simulink model "FSEA_Vehicle"  (R2026a)
settings: Solver=ode23tb  StopTime=5  FixedStep=.001  RelTol=1e-1
model workspace (MAT data in the model file):
  A_mu = 10
  B_reff = 8.386
  CONVERTER_DATA = [0 0.1 0.2 0.3 0.4 0.5 0.6 0.7 0.8 0.81 0.82 0.83 ... (63 elements, 21x3)]
  Cps = 2
  Cz = 7766.25
  DOWN_TABLE = [0 0 0 0 0 0 5 5 7.5 7.5 15 15 ... (30 elements, 6x5)]
  DOWN_TH_BP = [0 5 40 50 90 100]
  D_reff = 0.25826
  EMAP = [-40 215 245 264 264 267 267 267 267 267 -44 117 ... (110 elements, 10x11)]
  F0z = [6086.4 4324.8]
  F_reff = 0.07394
  F_zmax = 10000
  F_zmin = 100
  F_zo = 4000
  Kz = 48000
  MF : object (value not decoded)
  NCyl = 6
  NE_VEC = [800 1200 1600 2000 2400 2800 3200 3600 4000 4400 4800]
  Pstd = 101325
  Rair = 287
  SUS : object (value not decoded)
  TH_VEC = [0; 20; 30; 40; 50; 60; 70; 80; 90; 100]
  TWAITdn = 1.25
  TWAITup = 0.1
  Tin = [1 2 3 4 5 6 7 8 9 10 2 2 ... (20 elements, 10x2)]
  Tstd = 293.15
  UP_TABLE = [7.5 7.5 15 25 40 40 25 25 35 45 70 80 ... (30 elements, 6x5)]
  UP_TH_BP = [0 25 35 50 90 100]
  VEH : object (value not decoded)
  V_o = 16.7
  V_xlow = 1
  Vd = 0.00346
  WH : object (value not decoded)
  a = 1.515
  alpha_max = 1.5
  alpha_min = -1.5
  b = 1.504
  c_zo = 209651
  epsilon = 0.1
  f_air = [0 0 0 0 0 0 0 0 0 0 0 0 ... (256 elements, 16x16)]
  f_co = [0 0 0 0 0 0 0 0 0 0 0 0 ... (256 elements, 16x16)]
  f_co2 = [0 0 0 0 0 0 0 0 0 0 0 0 ... (256 elements, 16x16)]
  f_eff = [352.135682859 352.135682859 320.724378192 303.655312657 295.930136708 291.240087194 291.240271258 291.240312459 291.240275452 291.240198499 291.240100781 291.240018769 ... (256 elements, 16x16)]
  f_fuel = [0 0 0 0 0 0 0 0 0 0 0 0 ... (256 elements, 16x16)]
  f_hc = [0 0 0 0 0 0 0 0 0 0 0 0 ... (256 elements, 16x16)]
  f_nox = [0 0 0 0 0 0 0 0 0 0 0 0 ... (256 elements, 16x16)]
  f_pm = [0 0 0 0 0 0 0 0 0 0 0 0 ... (256 elements, 16x16)]
  f_susp_axl_bp = [1 2]
  f_susp_dz_bp = [-4 -0.14 -0.13 -0.12 -0.11 -0.1 -0.09 -0.08 -0.07 -0.06 -0.05 -0.04 ... (31 elements, 1x31)]
  f_susp_dzdot_bp = [-4 -0.14 -0.13 -0.12 -0.11 -0.1 -0.09 -0.08 -0.07 -0.06 -0.05 -0.04 ... (31 elements, 1x31)]
  f_susp_fmz = [-213379.591456 -28099.591456 -27619.591456 -27139.591456 -26659.591456 -26179.591456 -25699.591456 -25219.591456 -24739.591456 -24259.591456 -23779.591456 -23299.591456 ... (468968 elements, 31x31x61x2x4)]
  f_susp_geom = [-0.832564012244 0.043269987756 0.045538987756 0.047807987756 0.050076987756 0.052345987756 0.054614987756 0.056883987756 0.059152987756 0.061421987756 0.063690987756 0.065959987756 ... (11346 elements, 31x61x2x3)]
  f_susp_strgdelta_bp = [-0.523598775598 -0.506145483078 -0.488692190558 -0.471238898038 -0.453785605519 -0.436332312999 -0.418879020479 -0.401425727959 -0.383972435439 -0.366519142919 -0.349065850399 -0.331612557879 ... (61 elements, 1x61)]
  f_tbrake = [0 76.8593923996 105.140482948 131.533638111 157.926793274 176.658631717 176.65727296 176.656856686 176.656879077 176.657093756 176.657404516 176.65772406 ... (256 elements, 16x16)]
  f_tbrake_n_bpt = [0 649.519052838 912.419621844 1175.32019085 1438.22075986 1701.12132886 1964.02189787 2226.92246687 2489.82303588 2752.72360489 3015.62417389 3278.5247429 ... (16 elements, 1x16)]
  f_tbrake_t_bpt = [0 34.6410161514 61.0341713143 87.4273264773 113.82048164 140.213636803 166.606791966 192.999947129 219.393102292 245.786257455 272.179412618 298.572567781 ... (16 elements, 1x16)]
  f_texh = [766.752464599 766.752464599 786.17542386 801.679939032 884.591982581 910.574397722 910.571871054 910.570774534 910.570601632 910.570821151 910.571247242 910.571639815 ... (256 elements, 16x16)]
  f_twc_eff_co = [0.17 0.25 0.45 0.99 0.99 0.99 0.99]
  f_twc_eff_hc = [0.21 0.375 0.75 0.98 0.98 0.98 0.98]
  f_twc_eff_lam = [0.909090909 0.944055944 0.979020979 1 1.013986014 1.048951049 1.083916084]
  f_twc_eff_nox = [0.98 0.98 0.98 0.97 0.05 0.02 0]
  h = 0.134
  k_z = 50
  kappa_max = 1.5
  kappa_min = -1.5
  lam_Cx = 1
  lam_Cy = 1
  lam_Cz = 1
  lam_Ex = 1
  lam_Ey = 1
  lam_F_zo = 1
  lam_Hx = 1
  lam_Hy = 1
  lam_Kxkappa = 1
  lam_Kyalpha = 1
  lam_Kygamma = 1
  lam_Kzgamma = 1
  lam_Mr = 1
  lam_Mx = 1
  lam_My = 1
  lam_S = 1
  lam_VMx = 1
  lam_Vx = 1
  lam_Vy = 1
  lam_Vykappa = 1
  lam_muV = 0
  lam_mux = 1
  lam_muy = 1
  lam_t = 1
  lam_xalpha = 1
  lam_ykappa = 1
  numWheel = 4
  p_Cx1 = 1.579
  p_Cy1 = 1.3332
  p_Dx1 = 1.0422
  p_Dx2 = -0.08285
  p_Dx3 = 0
  p_Dy1 = 0.8784
  p_Dy2 = -0.06445
  p_Dy3 = 0
  p_Ex1 = 0.11185
  p_Ex2 = 0.3127
  p_Ex3 = 0
  p_Ex4 = 0.001603
  p_Ey1 = -0.8227
  p_Ey2 = -0.6062
  p_Ey3 = 0.09825
  p_Ey4 = -6.546
  p_Ey5 = 0
  p_Fz1 = 0.7098
  p_Hx1 = 0.00021585
  p_Hx2 = 0.0011538
  p_Hy1 = -0.0018043
  p_Hy2 = 0.003518
  p_Kx1 = 21.69
  p_Kx2 = 13.774
  p_Kx3 = -0.4119
  p_Ky1 = -15.314
  p_Ky2 = 1.7044
  p_Ky3 = 0.36986
  p_Ky4 = 1.9896
  p_Ky5 = 0
  p_Ky6 = -0.9004
  p_Ky7 = -0.2328
  p_Vx1 = 1.5973e-05
  p_Vx2 = 0.0001043
  p_Vy1 = -0.006642
  p_Vy2 = 0.03597
  p_Vy3 = -0.1621
  p_Vy4 = -0.4908
  p_pmx1 = 0
  p_px1 = -0.3489
  p_px2 = 0.382
  p_px3 = -0.09634
  p_px4 = 0.06447
  p_py1 = -0.6249
  p_py2 = -0.06535
  p_py3 = -0.1668
  p_py4 = 0.2834
  p_py5 = 0
  path : object (value not decoded)
  pio = 220000
  q_Fcx = 0
  q_Fz2 = 15.4
  q_Fzy = 0
  q_reo = 0.9974
  q_sx1 = -0.007764
  q_sx10 = 0.2824
  q_sx11 = 5.349
  q_sx12 = 0
  q_sx13 = 0
  q_sx14 = 0
  q_sx2 = 1.1915
  q_sx3 = 0.013948
  q_sx4 = 4.912
  q_sx5 = 1.02
  q_sx6 = 22.83
  q_sx7 = 0.7104
  q_sx8 = -0.023393
  q_sx9 = 0.6581
  q_sy1 = 0.00702
  q_sy2 = 0
  q_sy3 = 0.001515
  q_sy4 = 8.514e-05
  q_sy5 = 0
  q_sy6 = 0
  q_sy7 = 0.9008
  q_sy8 = -0.4089
  q_v1 = 0.0007742
  q_v2 = 0.04667
  r_Bx1 = 12.531
  r_Bx2 = 9.532
  r_Bx3 = 0
  r_By1 = 10.615
  r_By2 = 7.705
  r_By3 = 3.433e-06
  r_By4 = 0
  r_Cx1 = 1.019
  r_Cy1 = 1.0585
  r_Ex1 = -0.4487
  r_Ex2 = -0.4726
  r_Ey1 = 0.3132
  r_Ey2 = 7.63e-06
  r_Hx1 = 0.0002374
  r_Hy1 = 0.011646
  r_Hy2 = 7.63e-06
  r_Vy1 = 0.05654
  r_Vy2 = 7.63e-06
  r_Vy3 = 0
  r_Vy4 = 99.9
  r_Vy5 = 2
  r_Vy6 = 15.814
  r_o = 0.3135
  reqTmaxT = [nan 0.285774810084 0.647179872268 nan nan nan nan nan nan nan nan nan ... (168 elements, 21x8)]
  vehSpd = [0 2.77777777778 5.55555555556 8.33333333333 11.1111111111 13.8888888889 16.6666666667 19.4444444444 22.2222222222 25 27.7777777778 30.5555555556 ... (21 elements, 1x21)]
  vehWidth = 2
  w = 1
symbols that are objects in the model workspace (value not decoded): VEH
undefined symbols (not defined in the file or in its folder): InertFrm
libraries: sharedtransform x6, vehdynlibtirecommon x2, vehdynlibtire x2, autolibutils x2, autolibshared x2
(part 2 of 4)

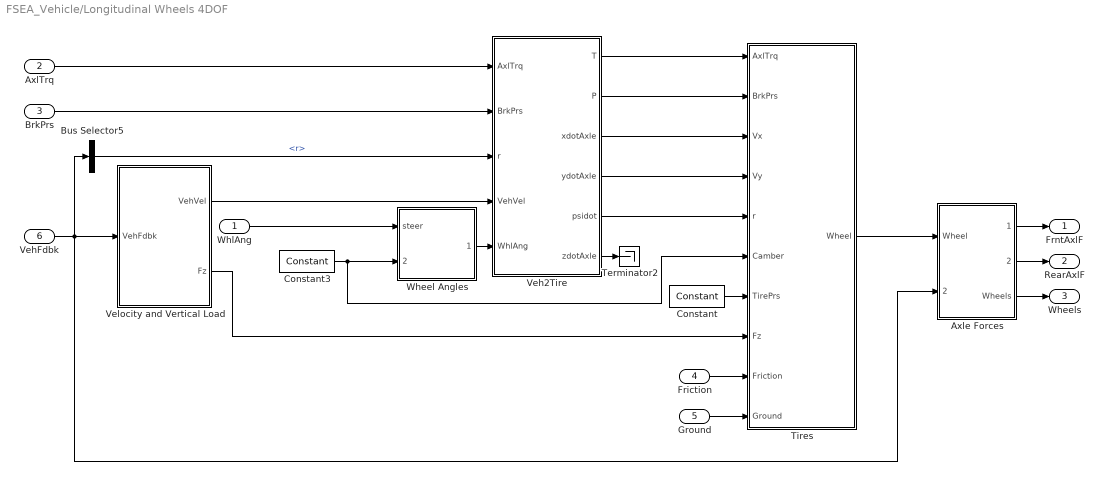
== system FSEA_Vehicle/Longitudinal Wheels 4DOF ==
  WhlAng : Inport
  AxlTrq : Inport  Port=2
  BrkPrs : Inport  Port=3
  Friction : Inport  Port=4  PortDimensions=4
  Ground : Inport  Port=5  PortDimensions=4
  VehFdbk : Inport  Port=6
  Axle Forces : Subsystem  Variant=on  VariantControlMode=label  LabelModeActiveChoice=1
  Bus Selector5 : BusSelector  OutputSignals=BdyFrm.Cg.AngVel.r
  Constant : vehdynlibtirecommon/Constant  const=220000  numWheels=4
  Constant3 : vehdynlibtirecommon/Constant  const=0  numWheels=4
  Terminator2 : Terminator
  Tires : Subsystem  Variant=on  VariantControlMode=label  VariantControl=Choice  LabelModeActiveChoice=0
  Veh2Tire : Subsystem
  Velocity and Vertical Load : Subsystem  Variant=on  VariantControlMode=label  LabelModeActiveChoice=1
  Wheel Angles : Subsystem
  FrntAxlF : Outport  Unit=N  VectorParamsAs1DForOutWhenUnconnected=off
  RearAxlF : Outport  Port=2  Unit=N  VectorParamsAs1DForOutWhenUnconnected=off
  Wheels : Outport  Port=3  VectorParamsAs1DForOutWhenUnconnected=off
  wires:
  Wheel Angles/1(WhlAngB) -> Veh2Tire/5(WhlAng)
  Constant/1 -> Tires/7(TirePrs)
  Constant3/1 -> Wheel Angles/2(camber), Tires/6(Camber)
  Veh2Tire/1(T) -> Tires/1(AxlTrq)
  Veh2Tire/2(P) -> Tires/2(BrkPrs)
  BrkPrs/1 -> Veh2Tire/2(BrkPrs)
  Veh2Tire/6(zdotAxle) -> Terminator2/1
  Veh2Tire/5(psidot) -> Tires/5(r)
  Velocity and Vertical Load/2(Fz) -> Tires/8(Fz)
  Velocity and Vertical Load/1(VehVel) -> Veh2Tire/4(VehVel)
  Axle Forces/1(FrntAxlF) -> FrntAxlF/1
  Axle Forces/2(RearAxlF) -> RearAxlF/1
  Tires/1(Wheel) -> Axle Forces/1(Wheel)
  Axle Forces/3(Wheels) -> Wheels/1
  VehFdbk/1 -> Axle Forces/2(VehFdbk), Bus Selector5/1, Velocity and Vertical Load/1(VehFdbk)
  Ground/1 -> Tires/10(Ground)
  WhlAng/1 -> Wheel Angles/1(steer)
  AxlTrq/1 -> Veh2Tire/1(AxlTrq)
  Friction/1 -> Tires/9(Friction)
  Bus Selector5/1 -> Veh2Tire/3(r)  "<r>"
  Veh2Tire/4(ydotAxle) -> Tires/4(Vy)
  Veh2Tire/3(xdotAxle) -> Tires/3(Vx)

== system FSEA_Vehicle/Vehicle Body 3DOF External Longitudinal Wheels ==
  WhlAng : Inport
  "FwF " : Inport  Port=2
  "FwR " : Inport  Port=3
  WindXYZ : Inport  Port=4
  Bicycle : Subsystem  VariantControl=0
  Dual : Subsystem  VariantControl=1
  " Info" : Outport  VectorParamsAs1DForOutWhenUnconnected=off

== system FSEA_Vehicle/Vehicle Signal Routing ==
  Info : Inport
  Ground : Inport  Port=2
  Dual Track Vehicle Signal Routing : Subsystem  VariantControl=1
  Single Track Vehicle Signal Routing : Subsystem  VariantControl=0
  VehFdbk : Outport

== system FSEA_Vehicle/Longitudinal Wheels 4DOF/Axle Forces ==
  note: 1) Add Subsystem or Model blocks as valid variant choices.
      | 2) You cannot connect blocks at this level. At simulation, connectivity is automatically
      | determined, based on the active variant and port name matching.
  Wheel : Inport
  VehFdbk : Inport  Port=2
  Bicycle : Subsystem  VariantControl=0
  Dual : Subsystem  VariantControl=1
  FrntAxlF : Outport  Unit=N  VectorParamsAs1DForOutWhenUnconnected=off
  RearAxlF : Outport  Port=2  Unit=N  VectorParamsAs1DForOutWhenUnconnected=off
  Wheels : Outport  Port=3

== system FSEA_Vehicle/Longitudinal Wheels 4DOF/Tires ==
  AxlTrq : Inport
  BrkPrs : Inport  Port=2
  Vx : Inport  Port=3
  Vy : Inport  Port=4
  r : Inport  Port=5
  Camber : Inport  Port=6
  TirePrs : Inport  Port=7
  Fz : Inport  Port=8
  Friction : Inport  Port=9
  Ground : Inport  Port=10
  Fiala : Subsystem  VariantControl=1
  MF : Subsystem  VariantControl=0
  Wheel : Outport

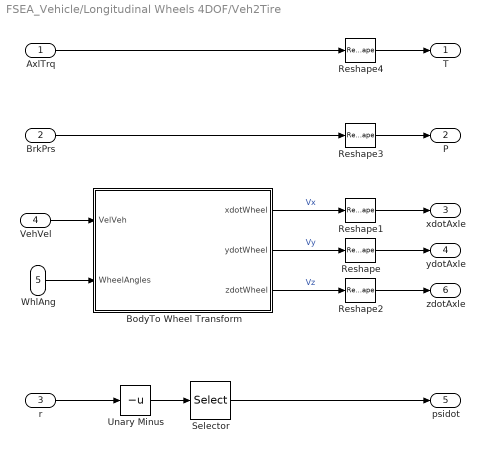
== system FSEA_Vehicle/Longitudinal Wheels 4DOF/Veh2Tire ==
  AxlTrq : Inport
  BrkPrs : Inport  Port=2
  r : Inport  Port=3
  VehVel : Inport  Port=4
  WhlAng : Inport  Port=5
  BodyTo Wheel Transform : Subsystem
  Reshape{,1..4} (5 alike) : Reshape
  Selector : Selector  InputPortWidth=1  IndexOptions=Index vector (dialog)  Indices=[1 1 1 1]  OutputSizes=1
  Unary Minus : UnaryMinus
  T : Outport  VectorParamsAs1DForOutWhenUnconnected=off
  P : Outport  Port=2  VectorParamsAs1DForOutWhenUnconnected=off
  xdotAxle : Outport  Port=3  VectorParamsAs1DForOutWhenUnconnected=off
  ydotAxle : Outport  Port=4  VectorParamsAs1DForOutWhenUnconnected=off
  psidot : Outport  Port=5  VectorParamsAs1DForOutWhenUnconnected=off
  zdotAxle : Outport  Port=6  VectorParamsAs1DForOutWhenUnconnected=off
  wires:
  BrkPrs/1 -> Reshape3/1
  AxlTrq/1 -> Reshape4/1
  BodyTo Wheel Transform/1(xdotWheel) -> Reshape1/1  "Vx"
  BodyTo Wheel Transform/2(ydotWheel) -> Reshape/1  "Vy"
  r/1 -> Unary Minus/1
  Reshape4/1 -> T/1
  VehVel/1 -> BodyTo Wheel Transform/1(VelVeh)
  BodyTo Wheel Transform/3(zdotWheel) -> Reshape2/1  "Vz"
  Unary Minus/1 -> Selector/1
  Reshape3/1 -> P/1
  WhlAng/1 -> BodyTo Wheel Transform/2(WheelAngles)
  Selector/1 -> psidot/1
  Reshape/1 -> ydotAxle/1
  Reshape1/1 -> xdotAxle/1
  Reshape2/1 -> zdotAxle/1

== system FSEA_Vehicle/Longitudinal Wheels 4DOF/Velocity and Vertical Load ==
  note: 1) Add Subsystem or Model blocks as valid variant choices.
      | 2) You cannot connect blocks at this level. At simulation, connectivity is automatically
      | determined, based on the active variant and port name matching.
  VehFdbk : Inport
  Bicycle : Subsystem  VariantControl=0
  Dual : Subsystem  VariantControl=1
  VehVel : Outport  VectorParamsAs1DForOutWhenUnconnected=off
  Fz : Outport  Port=2  PortDimensions=4  VectorParamsAs1DForOutWhenUnconnected=off

== system FSEA_Vehicle/Longitudinal Wheels 4DOF/Wheel Angles ==
  steer : Inport
  camber : Inport  Port=2
  Constant3 : Constant  Value=ones(1,4).*0
  Reshape : Reshape  OutputDimensionality=Row vector (2-D)
  Reshape1 : Reshape  OutputDimensionality=Row vector (2-D)
  Reshape2 : Reshape  OutputDimensionality=Row vector (2-D)
  Vector Concatenate3 : Concatenate  NumInputs=3  Mode=Multidimensional array
  WhlAngB : Outport  VectorParamsAs1DForOutWhenUnconnected=off
  wires:
  camber/1 -> Reshape1/1
  steer/1 -> Reshape/1
  Reshape2/1 -> Vector Concatenate3/2
  Reshape1/1 -> Vector Concatenate3/1
  Constant3/1 -> Reshape2/1
  Reshape/1 -> Vector Concatenate3/3
  Vector Concatenate3/1 -> WhlAngB/1

== system FSEA_Vehicle/Vehicle Body 3DOF External Longitudinal Wheels/Bicycle ==
  "FwF " : Inport
  "FwR " : Inport  Port=2
  WindXYZ : Inport  Port=3
  Terminator{,1..5} (6 alike) : Terminator
  Vehicle Body 3DOF Single Track : autolibshared/Vehicle Body 3DOF Single Track  trackMode=Single (bicycle)  inputMode=External forces  frontSteerMode=off  rearSteerMode=off  extFMode=off  htchFMode=off  extMMode=off  htchMMode=off  windMode=on  extTamb=off  muMode=off  extGndPlnElev=off  extGndPlnRoll=off  extGndPlnPitch=off  extGndPlnDCM=off  extXo=off  extxdoto=off  extYo=off  extydoto=off  extpsio=off  extro=off  aMode=2  NF=VEH.NumberOfWheelsPerAxle  NR=VEH.NumberOfWheelsPerAxle  m=VEH.Mass  a=VEH.FrontAxlePositionfromCG  b=VEH.RearAxlePositionfromCG  h=VEH.HeightCG  dh=1  hh=0.2  X_o=VEH.InitialLongPosition  xdot_o=VEH.InitialLongVel  d=0  hl=0  w=1.922.*[1 1]  CalphaMode=Constant  sigmaMode=on  sigma_f=.1  sigma_r=.1  Cy_f=15000  Cy_r=35000  Cy_f_data=[-9e3 9e3]  alpha_f_brk=[-.1 .1]  Fz_f_brk="[500\t1.555555555555556e+03\t2.611111111111111e+03\t3.666666666666667e+03\t4.722222222222223e+03\t5.777777777777777e+03\t6.833333333333333e+03\t7.888888888888889e+03\t8.944444444444445e+03\t10000]"  Cy_r_data=[-9e3 9e3]  alpha_r_brk=[-.1 .1]  Fz_r_brk="[500\t1.555555555555556e+03\t2.611111111111111e+03\t3.666666666666667e+03\t4.722222222222223e+03\t5.777777777777777e+03\t6.833333333333333e+03\t7.888888888888889e+03\t8.944444444444445e+03\t10000]"  Fznom=3800  Y_o=VEH.InitialLatPosition  ydot_o=VEH.InitialLatVel  Izz=VEH.YawMomentInertia  psi_o=VEH.InitialYawAngle  r_o=VEH.InitialYawRate  Af=VEH.FrontalArea  Cd=.3  Cl=.1  Cpm=.1  beta_w=[0 0.01:0.01:0.3]  Cs=ones(1,31).*0.3  Cym=[0 1e-6:0.01:0.3]  Pabs=101325  Tair=273  g=9.81  mu=1  GndPlnRoll=0  GndPlnPitch=0  GndPlnElev=0  xdot_tol=.1  Fxtire_sat=7e3*1e3  Fytire_sat=2e3*1e3  longOff=0  latOff=0  vertOff=VEH.HeightCG  wrapAng=off
  " Info" : Outport  VectorParamsAs1DForOutWhenUnconnected=off
  wires:
  "FwR "/1 -> Vehicle Body 3DOF Single Track/2
  "FwF "/1 -> Vehicle Body 3DOF Single Track/1
  Vehicle Body 3DOF Single Track/1 -> " Info"/1
  Vehicle Body 3DOF Single Track/6 -> Terminator/1
  Vehicle Body 3DOF Single Track/7 -> Terminator1/1
  WindXYZ/1 -> Vehicle Body 3DOF Single Track/3
  Vehicle Body 3DOF Single Track/4 -> Terminator2/1
  Vehicle Body 3DOF Single Track/5 -> Terminator3/1
  Vehicle Body 3DOF Single Track/2 -> Terminator4/1
  Vehicle Body 3DOF Single Track/3 -> Terminator5/1

== system FSEA_Vehicle/Vehicle Body 3DOF External Longitudinal Wheels/Dual ==
  WhlAng : Inport
  "FwF " : Inport  Port=2
  "FwR " : Inport  Port=3
  WindXYZ : Inport  Port=4
  Selector : Selector  InputPortWidth=4  IndexOptions=Index vector (dialog)  Indices=[1 2]  OutputSizes=1
  Terminator{,1..5} (6 alike) : Terminator
  Vehicle Body 3DOF Dual Track : autolibshared/Vehicle Body 3DOF Single Track  trackMode=Dual  inputMode=External forces  frontSteerMode=on  rearSteerMode=off  extFMode=off  htchFMode=off  extMMode=off  htchMMode=off  windMode=on  extTamb=off  muMode=off  extGndPlnElev=off  extGndPlnRoll=off  extGndPlnPitch=off  extGndPlnDCM=off  extXo=off  extxdoto=off  extYo=off  extydoto=off  extpsio=off  extro=off  aMode=2  NF=VEH.NumberOfWheelsPerAxle  NR=VEH.NumberOfWheelsPerAxle  m=310  a=0.775  b=0.775  h=0.289  dh=1  hh=0.2  X_o=VEH.InitialLongPosition  xdot_o=VEH.InitialLatVel  d=0  hl=0  w=[1.200, 1.150]  CalphaMode=Constant  sigmaMode=on  sigma_f=.1  sigma_r=.1  Cy_f=15000  Cy_r=35000  Cy_f_data=[-9e3 9e3]  alpha_f_brk=[-.1 .1]  Fz_f_brk="[500\t1.555555555555556e+03\t2.611111111111111e+03\t3.666666666666667e+03\t4.722222222222223e+03\t5.777777777777777e+03\t6.833333333333333e+03\t7.888888888888889e+03\t8.944444444444445e+03\t10000]"  Cy_r_data=[-9e3 9e3]  alpha_r_brk=[-.1 .1]  Fz_r_brk="[500\t1.555555555555556e+03\t2.611111111111111e+03\t3.666666666666667e+03\t4.722222222222223e+03\t5.777777777777777e+03\t6.833333333333333e+03\t7.888888888888889e+03\t8.944444444444445e+03\t10000]"  Fznom=3800  Y_o=VEH.InitialLatPosition  ydot_o=VEH.InitialLatVel  Izz=VEH.YawMomentInertia  psi_o=VEH.InitialYawAngle  r_o=VEH.InitialYawRate  Af=1  Cd=.3  Cl=.1  Cpm=.1  beta_w=[0 0.01:0.01:0.3]  Cs=ones(1,31).*0.3  Cym=[0 1e-6:0.001:0.03]  Pabs=101325  Tair=273  g=9.81  mu=1  GndPlnRoll=0  GndPlnPitch=0  GndPlnElev=0  xdot_tol=.01  Fxtire_sat=7e3*1e3  Fytire_sat=2e3*1e3  longOff=0  latOff=0  vertOff=VEH.HeightCG  wrapAng=on
  " Info" : Outport  VectorParamsAs1DForOutWhenUnconnected=off
  wires:
  Vehicle Body 3DOF Dual Track/1 -> " Info"/1
  Vehicle Body 3DOF Dual Track/2 -> Terminator4/1
  Vehicle Body 3DOF Dual Track/3 -> Terminator5/1
  Vehicle Body 3DOF Dual Track/6 -> Terminator1/1
  Vehicle Body 3DOF Dual Track/4 -> Terminator2/1
  Vehicle Body 3DOF Dual Track/5 -> Terminator3/1
  Vehicle Body 3DOF Dual Track/7 -> Terminator/1
  WindXYZ/1 -> Vehicle Body 3DOF Dual Track/4
  WhlAng/1 -> Selector/1
  Selector/1 -> Vehicle Body 3DOF Dual Track/1
  "FwF "/1 -> Vehicle Body 3DOF Dual Track/2
  "FwR "/1 -> Vehicle Body 3DOF Dual Track/3

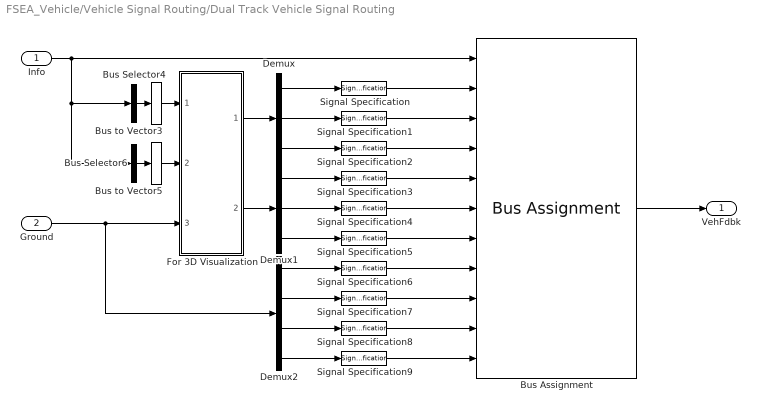
== system FSEA_Vehicle/Vehicle Signal Routing/Dual Track Vehicle Signal Routing ==
  Info : Inport
  Ground : Inport  Port=2
  Bus Assignment : BusAssignment  AssignedSignals=InertFrm.Cg.Ang.phi,InertFrm.Cg.Ang.theta,InertFrm.Cg.Ang.psi,InertFrm.Geom.Disp.X,InertFrm.Geom.Disp.Y,InertFrm.Geom.Disp.Z,InertFrm.FrntAxl.Lft.Disp.Z,InertFrm.FrntAxl.Rght.Disp.Z,InertFrm.RearAxl.Lft.Disp.Z,InertFrm.RearAxl.Rght.Disp.Z
  Bus Selector4 : BusSelector  OutputSignals=InertFrm.Cg.Ang.phi,InertFrm.Cg.Ang.theta,InertFrm.Cg.Ang.psi  OutputAsBus=on
  Bus Selector6 : BusSelector  OutputSignals=InertFrm.Geom.Disp.X,InertFrm.Geom.Disp.Y,InertFrm.Geom.Disp.Z  OutputAsBus=on
  Bus to Vector3 : BusToVector
  Bus to Vector5 : BusToVector
  Demux : Demux  Outputs=3
  Demux1 : Demux  Outputs=3
  Demux2 : Demux
  For 3D Visualization : MATLAB Function  TreatAsAtomicUnit=on  mask{trackW=VEH.TrackWidth, wheelB=VEH.FrontAxlePositionfromCG+VEH.RearAxlePositionfromCG}
      mask prompts: trackW "Vehicle track width, trackW [m]:"; wheelB "Vehicle wheelbase, wheelB [m]:"
      mask help: This block converts wheel ground height information into estimates of vehicle pitch, roll angles and vertical height in order to help in the visualization 3DOF based simulations with changes in terrain. Note that the resulting signals are only used as a visualization aid and do not account for the physical affects of the vehicle interacting with variable terrain or changes in orientation.
  Signal Specification : SignalSpecification  Unit=rad
  Signal Specification1 : SignalSpecification  Unit=rad
  Signal Specification2 : SignalSpecification  Unit=rad
  Signal Specification{3..9} (7 alike) : SignalSpecification  Unit=m
  VehFdbk : Outport  VectorParamsAs1DForOutWhenUnconnected=off
  wires:
  Info/1 -> Bus Selector4/1, Bus Selector6/1, Bus Assignment/1
  Bus to Vector3/1 -> For 3D Visualization/1(angleIn)
  For 3D Visualization/1(angles) -> Demux/1
  Bus Selector6/1 -> Bus to Vector5/1
  Ground/1 -> Demux2/1, For 3D Visualization/3(Ground)
  For 3D Visualization/2(GeomXYZ) -> Demux1/1
  Bus to Vector5/1 -> For 3D Visualization/2(GemoXYZIn)
  Bus Selector4/1 -> Bus to Vector3/1
  Demux/2 -> Signal Specification1/1
  Demux/1 -> Signal Specification/1
  Demux/3 -> Signal Specification2/1
  Demux1/1 -> Signal Specification3/1
  Demux1/2 -> Signal Specification4/1
  Demux1/3 -> Signal Specification5/1
  Bus Assignment/1 -> VehFdbk/1
  Signal Specification/1 -> Bus Assignment/2
  Signal Specification1/1 -> Bus Assignment/3
  Signal Specification2/1 -> Bus Assignment/4
  Signal Specification3/1 -> Bus Assignment/5
  Signal Specification4/1 -> Bus Assignment/6
  Signal Specification5/1 -> Bus Assignment/7
  Demux2/3 -> Signal Specification8/1
  Demux2/2 -> Signal Specification7/1
  Demux2/1 -> Signal Specification6/1
  Demux2/4 -> Signal Specification9/1
  Signal Specification6/1 -> Bus Assignment/8
  Signal Specification7/1 -> Bus Assignment/9
  Signal Specification8/1 -> Bus Assignment/10
  Signal Specification9/1 -> Bus Assignment/11

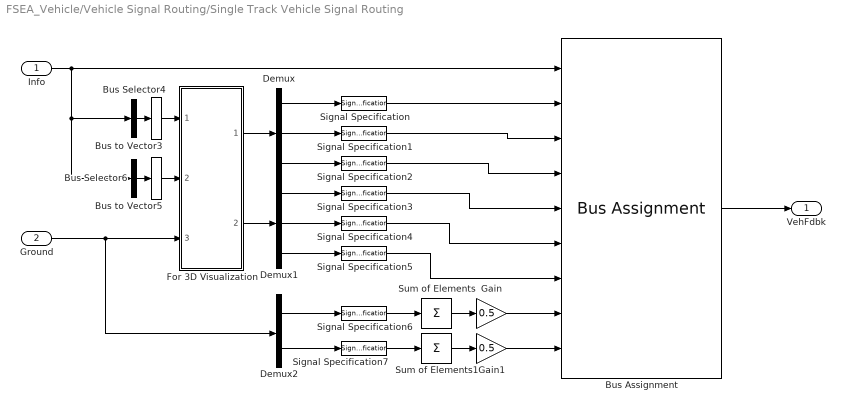
== system FSEA_Vehicle/Vehicle Signal Routing/Single Track Vehicle Signal Routing ==
  Info : Inport
  Ground : Inport  Port=2
  Bus Assignment : BusAssignment  AssignedSignals=InertFrm.Cg.Ang.phi,InertFrm.Cg.Ang.theta,InertFrm.Cg.Ang.psi,InertFrm.Geom.Disp.X,InertFrm.Geom.Disp.Y,InertFrm.Geom.Disp.Z,InertFrm.FrntAxl.Disp.Z,InertFrm.RearAxl.Disp.Z
  Bus Selector4 : BusSelector  OutputSignals=InertFrm.Cg.Ang.phi,InertFrm.Cg.Ang.theta,InertFrm.Cg.Ang.psi  OutputAsBus=on
  Bus Selector6 : BusSelector  OutputSignals=InertFrm.Geom.Disp.X,InertFrm.Geom.Disp.Y,InertFrm.Geom.Disp.Z  OutputAsBus=on
  Bus to Vector3 : BusToVector
  Bus to Vector5 : BusToVector
  Demux : Demux  Outputs=3
  Demux1 : Demux  Outputs=3
  Demux2 : Demux  Outputs=[2 2]
  For 3D Visualization : MATLAB Function  TreatAsAtomicUnit=on  mask{trackW=VEH.TrackWidth, wheelB=VEH.FrontAxlePositionfromCG+VEH.RearAxlePositionfromCG}
      mask prompts: trackW "Vehicle track width, trackW [m]:"; wheelB "Vehicle wheelbase, wheelB [m]:"
      mask help: This block converts wheel ground height information into estimates of vehicle pitch, roll angles and vertical height in order to help in the visualization 3DOF based simulations with changes in terrain. Note that the resulting signals are only used as a visualization aid and do not account for the physical affects of the vehicle interacting with variable terrain or changes in orientation.
  Gain : Gain  Gain=0.5
  Gain1 : Gain  Gain=0.5
  Signal Specification : SignalSpecification  Unit=rad
  Signal Specification1 : SignalSpecification  Unit=rad
  Signal Specification2 : SignalSpecification  Unit=rad
  Signal Specification{3..7} (5 alike) : SignalSpecification  Unit=m
  Sum of Elements : Sum  Inputs=+
  Sum of Elements1 : Sum  Inputs=+
  VehFdbk : Outport  VectorParamsAs1DForOutWhenUnconnected=off
  wires:
  Demux2/1 -> Signal Specification6/1
  Demux2/2 -> Signal Specification7/1
  Signal Specification5/1 -> Bus Assignment/7
  Signal Specification4/1 -> Bus Assignment/6
  Signal Specification3/1 -> Bus Assignment/5
  Signal Specification2/1 -> Bus Assignment/4
  Signal Specification1/1 -> Bus Assignment/3
  Signal Specification/1 -> Bus Assignment/2
  Bus Assignment/1 -> VehFdbk/1
  Demux1/3 -> Signal Specification5/1
  Demux1/2 -> Signal Specification4/1
  Demux1/1 -> Signal Specification3/1
  Demux/3 -> Signal Specification2/1
  Demux/1 -> Signal Specification/1
  Demux/2 -> Signal Specification1/1
  Bus Selector4/1 -> Bus to Vector3/1
  Bus to Vector5/1 -> For 3D Visualization/2(GemoXYZIn)
  For 3D Visualization/2(GeomXYZ) -> Demux1/1
  Ground/1 -> For 3D Visualization/3(Ground), Demux2/1
  Bus Selector6/1 -> Bus to Vector5/1
  For 3D Visualization/1(angles) -> Demux/1
  Bus to Vector3/1 -> For 3D Visualization/1(angleIn)
  Info/1 -> Bus Assignment/1, Bus Selector6/1, Bus Selector4/1
  Signal Specification6/1 -> Sum of Elements/1
  Gain/1 -> Bus Assignment/8
  Sum of Elements/1 -> Gain/1
  Sum of Elements1/1 -> Gain1/1
  Gain1/1 -> Bus Assignment/9
  Signal Specification7/1 -> Sum of Elements1/1

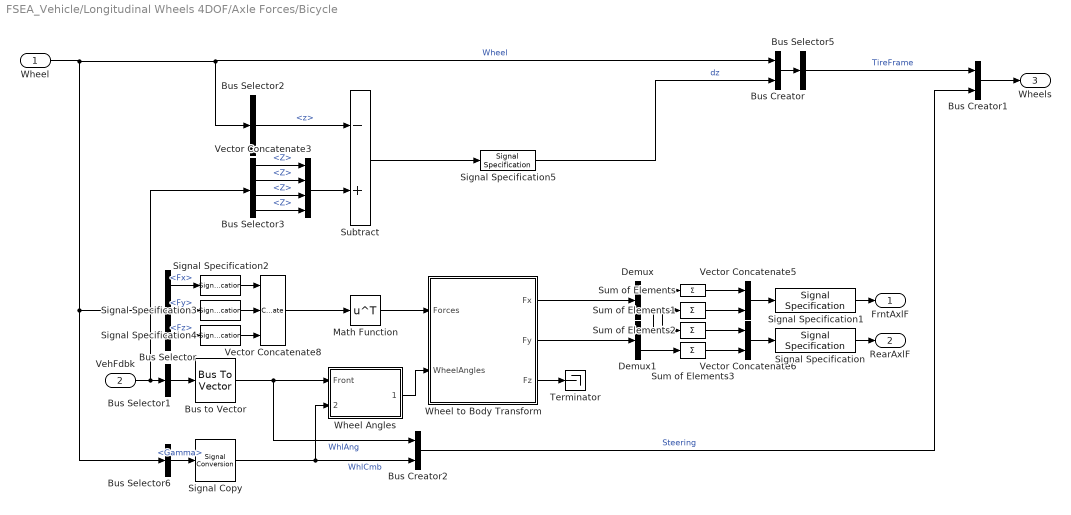
== system FSEA_Vehicle/Longitudinal Wheels 4DOF/Axle Forces/Bicycle ==
  Wheel : Inport
  VehFdbk : Inport  Port=2
  Bus Creator : BusCreator  Inputs=2
  Bus Creator1 : BusCreator  Inputs=2
  Bus Creator2 : BusCreator  Inputs=2
  Bus Selector : BusSelector  OutputSignals=Fx,Fy,Fz
  Bus Selector1 : BusSelector  OutputSignals=BdyFrm.FrntAxl.Steer.WhlAngFL,BdyFrm.FrntAxl.Steer.WhlAngFR,BdyFrm.RearAxl.Steer.WhlAngRL,BdyFrm.RearAxl.Steer.WhlAngRR  OutputAsBus=on
  Bus Selector2 : BusSelector  OutputSignals=z
  Bus Selector3 : BusSelector  OutputSignals=InertFrm.FrntAxl.Disp.Z,InertFrm.FrntAxl.Disp.Z,InertFrm.RearAxl.Disp.Z,InertFrm.RearAxl.Disp.Z
  Bus Selector5 : BusSelector  OutputSignals=Wheel.AxlTrq,Wheel.Omega,Wheel.Fx,Wheel.Fy,Wheel.Fz,Wheel.Mx,Wheel.My,Wheel.Mz,Wheel.Vx,Wheel.Vy,Wheel.Re,dz,Wheel.Kappa,Wheel.Alpha,Wheel.a,Wheel.b,Wheel.Gamma,Wheel.psidot,Wheel.BrkTrq,Wheel.BrkPrs,Wheel.z,Wheel.zdot,Wheel.Gnd,Wheel.GndFz,Wheel.Prs  OutputAsBus=on
  Bus Selector6 : BusSelector  OutputSignals=Gamma
  Bus to Vector : BusToVector
  Demux : Demux  Outputs=[2,2]
  Demux1 : Demux  Outputs=[2,2]
  Math Function : Math  Operator=transpose  SignedPower=on
  Signal Copy : SignalConversion  OverrideOpt=off
  Signal Specification : SignalSpecification  Unit=N
  Signal Specification1 : SignalSpecification  Unit=N
  Signal Specification2 : SignalSpecification  Dimensions=4
  Signal Specification3 : SignalSpecification  Dimensions=4
  Signal Specification4 : SignalSpecification  Dimensions=4
  Signal Specification5 : SignalSpecification  Unit=m
  Subtract : Sum  Inputs=-+
  Sum of Elements{,1..3} (4 alike) : Sum  Inputs=+
  Terminator : Terminator
  Vector Concatenate3 : Concatenate  NumInputs=4
  Vector Concatenate5 : Concatenate  Mode=Multidimensional array  ConcatenateDimension=2
  Vector Concatenate6 : Concatenate  Mode=Multidimensional array  ConcatenateDimension=2
  Vector Concatenate8 : Concatenate  NumInputs=3  Mode=Multidimensional array  ConcatenateDimension=2
  Wheel Angles : Subsystem
  Wheel to Body Transform : Subsystem
  FrntAxlF : Outport  Unit=N  VectorParamsAs1DForOutWhenUnconnected=off
  RearAxlF : Outport  Port=2  Unit=N  VectorParamsAs1DForOutWhenUnconnected=off
  Wheels : Outport  Port=3
  wires:
  Bus Selector/3 -> Signal Specification4/1  "<Fz>"
  Vector Concatenate6/1 -> Signal Specification/1
  Signal Specification2/1 -> Vector Concatenate8/1
  Vector Concatenate8/1 -> Math Function/1
  Demux/1 -> Sum of Elements/1
  Wheel to Body Transform/3(Fz) -> Terminator/1
  Signal Specification4/1 -> Vector Concatenate8/3
  Demux1/2 -> Sum of Elements3/1
  Demux1/1 -> Sum of Elements1/1
  Math Function/1 -> Wheel to Body Transform/1(Forces)
  Demux/2 -> Sum of Elements2/1
  Wheel to Body Transform/1(Fx) -> Demux/1
  Vector Concatenate5/1 -> Signal Specification1/1
  Signal Specification3/1 -> Vector Concatenate8/2
  Bus Selector/1 -> Signal Specification2/1  "<Fx>"
  Bus Selector/2 -> Signal Specification3/1  "<Fy>"
  Signal Specification/1 -> RearAxlF/1
  Signal Specification1/1 -> FrntAxlF/1
  Bus Selector1/1 -> Bus to Vector/1
  Sum of Elements/1 -> Vector Concatenate5/1
  Sum of Elements1/1 -> Vector Concatenate5/2
  Sum of Elements2/1 -> Vector Concatenate6/1
  Sum of Elements3/1 -> Vector Concatenate6/2
  Bus Selector2/1 -> Subtract/1  "<z>"
  Signal Specification5/1 -> Bus Creator/2  "dz"
  Vector Concatenate3/1 -> Subtract/2
  Subtract/1 -> Signal Specification5/1
  Bus Creator/1 -> Bus Selector5/1
  Bus Selector3/2 -> Vector Concatenate3/2  "<Z>"
  Bus Selector3/1 -> Vector Concatenate3/1  "<Z>"
  VehFdbk/1 -> Bus Selector3/1, Bus Selector1/1
  Bus Selector3/3 -> Vector Concatenate3/3  "<Z>"
  Bus Selector3/4 -> Vector Concatenate3/4  "<Z>"
  Bus Creator2/1 -> Bus Creator1/2  "Steering"
  Bus to Vector/1 -> Wheel Angles/1(Front), Bus Creator2/1  "WhlAng"
  Signal Copy/1 -> Wheel Angles/2(Camber), Bus Creator2/2  "WhlCmb"
  Bus Creator1/1 -> Wheels/1
  Bus Selector5/1 -> Bus Creator1/1  "TireFrame"
  Bus Selector6/1 -> Signal Copy/1  "<Gamma>"
  Wheel/1 -> Bus Selector6/1, Bus Selector/1, Bus Selector2/1, Bus Creator/1  "Wheel"
  Wheel Angles/1(Vehicle) -> Wheel to Body Transform/2(WheelAngles)
  Wheel to Body Transform/2(Fy) -> Demux1/1

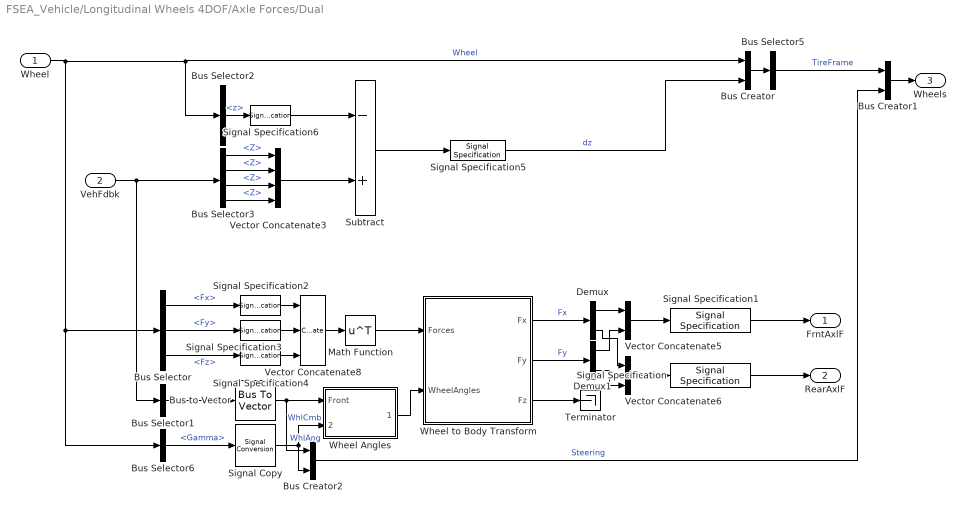
== system FSEA_Vehicle/Longitudinal Wheels 4DOF/Axle Forces/Dual ==
  Wheel : Inport
  VehFdbk : Inport  Port=2
  Bus Creator : BusCreator  Inputs=2
  Bus Creator1 : BusCreator  Inputs=2
  Bus Creator2 : BusCreator  Inputs=2
  Bus Selector : BusSelector  OutputSignals=Fx,Fy,Fz
  Bus Selector1 : BusSelector  OutputSignals=BdyFrm.FrntAxl.Steer.WhlAngFL,BdyFrm.FrntAxl.Steer.WhlAngFR,BdyFrm.RearAxl.Steer.WhlAngRL,BdyFrm.RearAxl.Steer.WhlAngRR  OutputAsBus=on
  Bus Selector2 : BusSelector  OutputSignals=z
  Bus Selector3 : BusSelector  OutputSignals=InertFrm.FrntAxl.Lft.Disp.Z,InertFrm.FrntAxl.Rght.Disp.Z,InertFrm.RearAxl.Lft.Disp.Z,InertFrm.RearAxl.Rght.Disp.Z
  Bus Selector5 : BusSelector  OutputSignals=Wheel.AxlTrq,Wheel.Omega,Wheel.Fx,Wheel.Fy,Wheel.Fz,Wheel.Mx,Wheel.My,Wheel.Mz,Wheel.Vx,Wheel.Vy,Wheel.Re,dz,Wheel.Kappa,Wheel.Alpha,Wheel.a,Wheel.b,Wheel.Gamma,Wheel.psidot,Wheel.BrkTrq,Wheel.BrkPrs,Wheel.z,Wheel.zdot,Wheel.Gnd,Wheel.GndFz,Wheel.Prs  OutputAsBus=on
  Bus Selector6 : BusSelector  OutputSignals=Gamma
  Bus to Vector : BusToVector
  Demux : Demux  Outputs=[2,2]
  Demux1 : Demux  Outputs=[2,2]
  Math Function : Math  Operator=transpose  SignedPower=on
  Signal Copy : SignalConversion  OverrideOpt=off
  Signal Specification : SignalSpecification  Unit=N
  Signal Specification1 : SignalSpecification  Unit=N
  Signal Specification{2..4,6} (4 alike) : SignalSpecification  Dimensions=4
  Signal Specification5 : SignalSpecification  Unit=m
  Subtract : Sum  Inputs=-+
  Terminator : Terminator
  Vector Concatenate3 : Concatenate  NumInputs=4
  Vector Concatenate5 : Concatenate  Mode=Multidimensional array  ConcatenateDimension=2
  Vector Concatenate6 : Concatenate  Mode=Multidimensional array  ConcatenateDimension=2
  Vector Concatenate8 : Concatenate  NumInputs=3  Mode=Multidimensional array  ConcatenateDimension=2
  Wheel Angles : Subsystem
  Wheel to Body Transform : Subsystem
  FrntAxlF : Outport  Unit=N  VectorParamsAs1DForOutWhenUnconnected=off
  RearAxlF : Outport  Port=2  Unit=N  VectorParamsAs1DForOutWhenUnconnected=off
  Wheels : Outport  Port=3
  wires:
  Bus Selector1/1 -> Bus to Vector/1
  Signal Specification1/1 -> FrntAxlF/1
  Signal Specification/1 -> RearAxlF/1
  Signal Specification3/1 -> Vector Concatenate8/2
  Math Function/1 -> Wheel to Body Transform/1(Forces)
  Signal Specification4/1 -> Vector Concatenate8/3
  Wheel to Body Transform/3(Fz) -> Terminator/1
  Vector Concatenate8/1 -> Math Function/1
  Signal Specification2/1 -> Vector Concatenate8/1
  VehFdbk/1 -> Bus Selector3/1, Bus Selector1/1
  Wheel/1 -> Bus Selector6/1, Bus Selector/1, Bus Creator/1, Bus Selector2/1  "Wheel"
  Bus Selector3/1 -> Vector Concatenate3/1  "<Z>"
  Subtract/1 -> Signal Specification5/1
  Vector Concatenate3/1 -> Subtract/2
  Bus Selector3/2 -> Vector Concatenate3/2  "<Z>"
  Bus Selector3/3 -> Vector Concatenate3/3  "<Z>"
  Signal Specification5/1 -> Bus Creator/2  "dz"
  Bus Selector2/1 -> Signal Specification6/1  "<z>"
  Bus Selector3/4 -> Vector Concatenate3/4  "<Z>"
  Bus Creator/1 -> Bus Selector5/1
  Bus Creator1/1 -> Wheels/1
  Signal Copy/1 -> Wheel Angles/2(Camber), Bus Creator2/2  "WhlCmb"
  Bus Creator2/1 -> Bus Creator1/2  "Steering"
  Bus Selector5/1 -> Bus Creator1/1  "TireFrame"
  Bus Selector/1 -> Signal Specification2/1  "<Fx>"
  Bus Selector/2 -> Signal Specification3/1  "<Fy>"
  Bus Selector/3 -> Signal Specification4/1  "<Fz>"
  Bus Selector6/1 -> Signal Copy/1  "<Gamma>"
  Bus to Vector/1 -> Wheel Angles/1(Front), Bus Creator2/1  "WhlAng"
  Signal Specification6/1 -> Subtract/1
  Wheel Angles/1(Vehicle) -> Wheel to Body Transform/2(WheelAngles)
  Vector Concatenate6/1 -> Signal Specification/1
  Wheel to Body Transform/2(Fy) -> Demux1/1  "Fy"
  Demux1/2 -> Vector Concatenate6/2
  Vector Concatenate5/1 -> Signal Specification1/1
  Wheel to Body Transform/1(Fx) -> Demux/1  "Fx"
  Demux1/1 -> Vector Concatenate5/2
  Demux/2 -> Vector Concatenate6/1
  Demux/1 -> Vector Concatenate5/1
